simulink model "gm_comm8qamtxrxhdl"  (R2025b)
settings: Solver=FixedStepDiscrete  StartTime=0.0  StopTime=20000*qam_params.symbolPeriod  RelTol=1e-3
PreLoadFcn:
  | qam_params = comm8qamtxrxhdl_init;
InitFcn:
  | qam_params = comm8qamtxrxhdl_init;
libraries: simulink x16, hdlmdlgenlib x7, hdlsllib x7, commchan3 x1, commrflib2 x1, dspsigops x1, dsphdlsigops2 x1, dspmlti4 x1, commdigbbndam3 x1, commsequence2 x1
(part 3 of 3)

== system gm_comm8qamtxrxhdl/QAM Rx HDL/Coarse Frequency Offset Correction/Frequency Offset Estimation/Iteration ==
  xin : Inport  OutDataTypeStr=fixdt(1, 17, 13)  SampleTime=5e-07
  yin : Inport  Port=2  OutDataTypeStr=fixdt(1, 17, 13)  SampleTime=5e-07
  zin : Inport  Port=3  OutDataTypeStr=fixdt(1, 19, 18)  SampleTime=5e-07
  lut_value : Inport  Port=4  OutDataTypeStr=fixdt(0, 16, 18)  SampleTime=5e-07
  idx : Inport  Port=5  OutDataTypeStr=fixdt(0, 4, 0)  SampleTime=5e-07
  MuxX : Switch  Criteria=u2 ~= 0  Threshold="fi(0,0,1,0,\"hex\",\"0\")"  OutDataTypeStr=fixdt(1, 17, 13)  SampleTime=5e-07  SaturateOnIntegerOverflow=off  InputSameDT=off
  MuxY : Switch  Criteria=u2 ~= 0  Threshold="fi(0,0,1,0,\"hex\",\"0\")"  OutDataTypeStr=fixdt(1, 17, 13)  SampleTime=5e-07  SaturateOnIntegerOverflow=off  InputSameDT=off
  MuxZ : Switch  Criteria=u2 ~= 0  Threshold="fi(0,0,1,0,\"hex\",\"0\")"  OutDataTypeStr=fixdt(1, 19, 18)  SampleTime=5e-07  SaturateOnIntegerOverflow=off  InputSameDT=off
  XAdder : Sum  OutDataTypeStr=fixdt(1, 17, 13)  SampleTime=5e-07
  XSubtractor : Sum  Inputs=+-  OutDataTypeStr=fixdt(1, 17, 13)  AccumDataTypeStr=fixdt(1, 17, 13)  SampleTime=5e-07
  YAdder : Sum  OutDataTypeStr=fixdt(1, 17, 13)  SampleTime=5e-07
  YSub : Sum  Inputs=+-  OutDataTypeStr=fixdt(1, 17, 13)  AccumDataTypeStr=fixdt(1, 17, 13)  SampleTime=5e-07
  ZAdder : Sum  OutDataTypeStr=fixdt(1, 19, 18)  SampleTime=5e-07
  ZSub : Sum  Inputs=+-  OutDataTypeStr=fixdt(1, 19, 18)  AccumDataTypeStr=fixdt(1, 19, 18)  SampleTime=5e-07
  compare : simulink/Logic and Bit Operations/Compare To Constant  relop=<  const=double(0)  OutDataTypeStr=boolean
  dynamic_shift : ArithShift  BitShiftNumberSource=Input port  BitShiftDirection=Right
      settings: InputPortMap=u0,p1
  dynamic_shift1 : ArithShift  BitShiftNumberSource=Input port  BitShiftDirection=Right
      settings: InputPortMap=u0,p1
  xout : Outport  OutDataTypeStr=fixdt(1, 17, 13)  SampleTime=5e-07
  yout : Outport  Port=2  OutDataTypeStr=fixdt(1, 17, 13)  SampleTime=5e-07
  zout : Outport  Port=3  OutDataTypeStr=fixdt(1, 19, 18)  SampleTime=5e-07
  wires:
  yin/1 -> YSub/1, YAdder/1, dynamic_shift1/1, compare/1
  xin/1 -> XAdder/1, XSubtractor/1, dynamic_shift/1
  dynamic_shift1/1 -> XAdder/2, XSubtractor/2
  idx/1 -> dynamic_shift1/2, dynamic_shift/2
  lut_value/1 -> ZAdder/2, ZSub/2
  dynamic_shift/1 -> YSub/2, YAdder/2
  YAdder/1 -> MuxY/1
  zin/1 -> ZAdder/1, ZSub/1
  YSub/1 -> MuxY/3
  XSubtractor/1 -> MuxX/1
  compare/1 -> MuxZ/2, MuxY/2, MuxX/2
  XAdder/1 -> MuxX/3
  ZSub/1 -> MuxZ/1
  ZAdder/1 -> MuxZ/3
  MuxY/1 -> yout/1
  MuxX/1 -> xout/1
  MuxZ/1 -> zout/1

== system gm_comm8qamtxrxhdl/QAM Rx HDL/Coarse Frequency Offset Correction/Frequency Offset Estimation/Iteration1 ==
  xin : Inport  OutDataTypeStr=fixdt(1, 17, 13)  SampleTime=5e-07
  yin : Inport  Port=2  OutDataTypeStr=fixdt(1, 17, 13)  SampleTime=5e-07
  zin : Inport  Port=3  OutDataTypeStr=fixdt(1, 19, 18)  SampleTime=5e-07
  lut_value : Inport  Port=4  OutDataTypeStr=fixdt(0, 16, 18)  SampleTime=5e-07
  idx : Inport  Port=5  OutDataTypeStr=fixdt(0, 4, 0)  SampleTime=5e-07
  MuxX : Switch  Criteria=u2 ~= 0  Threshold="fi(0,0,1,0,\"hex\",\"0\")"  OutDataTypeStr=fixdt(1, 17, 13)  SampleTime=5e-07  SaturateOnIntegerOverflow=off  InputSameDT=off
  MuxY : Switch  Criteria=u2 ~= 0  Threshold="fi(0,0,1,0,\"hex\",\"0\")"  OutDataTypeStr=fixdt(1, 17, 13)  SampleTime=5e-07  SaturateOnIntegerOverflow=off  InputSameDT=off
  MuxZ : Switch  Criteria=u2 ~= 0  Threshold="fi(0,0,1,0,\"hex\",\"0\")"  OutDataTypeStr=fixdt(1, 19, 18)  SampleTime=5e-07  SaturateOnIntegerOverflow=off  InputSameDT=off
  XAdder : Sum  OutDataTypeStr=fixdt(1, 17, 13)  SampleTime=5e-07
  XSubtractor : Sum  Inputs=+-  OutDataTypeStr=fixdt(1, 17, 13)  AccumDataTypeStr=fixdt(1, 17, 13)  SampleTime=5e-07
  YAdder : Sum  OutDataTypeStr=fixdt(1, 17, 13)  SampleTime=5e-07
  YSub : Sum  Inputs=+-  OutDataTypeStr=fixdt(1, 17, 13)  AccumDataTypeStr=fixdt(1, 17, 13)  SampleTime=5e-07
  ZAdder : Sum  OutDataTypeStr=fixdt(1, 19, 18)  SampleTime=5e-07
  ZSub : Sum  Inputs=+-  OutDataTypeStr=fixdt(1, 19, 18)  AccumDataTypeStr=fixdt(1, 19, 18)  SampleTime=5e-07
  compare : simulink/Logic and Bit Operations/Compare To Constant  relop=<  const=double(0)  OutDataTypeStr=boolean
  dynamic_shift : ArithShift  BitShiftNumberSource=Input port  BitShiftDirection=Right
      settings: InputPortMap=u0,p1
  dynamic_shift1 : ArithShift  BitShiftNumberSource=Input port  BitShiftDirection=Right
      settings: InputPortMap=u0,p1
  xout : Outport  OutDataTypeStr=fixdt(1, 17, 13)  SampleTime=5e-07
  yout : Outport  Port=2  OutDataTypeStr=fixdt(1, 17, 13)  SampleTime=5e-07
  zout : Outport  Port=3  OutDataTypeStr=fixdt(1, 19, 18)  SampleTime=5e-07
  wires:
  yin/1 -> YAdder/1, YSub/1, dynamic_shift1/1, compare/1
  xin/1 -> XSubtractor/1, XAdder/1, dynamic_shift/1
  idx/1 -> dynamic_shift/2, dynamic_shift1/2
  zin/1 -> ZSub/1, ZAdder/1
  dynamic_shift/1 -> YSub/2, YAdder/2
  ZSub/1 -> MuxZ/1
  dynamic_shift1/1 -> XSubtractor/2, XAdder/2
  lut_value/1 -> ZSub/2, ZAdder/2
  ZAdder/1 -> MuxZ/3
  YAdder/1 -> MuxY/1
  compare/1 -> MuxX/2, MuxY/2, MuxZ/2
  YSub/1 -> MuxY/3
  XSubtractor/1 -> MuxX/1
  XAdder/1 -> MuxX/3
  MuxZ/1 -> zout/1
  MuxY/1 -> yout/1
  MuxX/1 -> xout/1

== system gm_comm8qamtxrxhdl/QAM Rx HDL/Coarse Frequency Offset Correction/Frequency Offset Estimation/Iteration2 ==
  xin : Inport  OutDataTypeStr=fixdt(1, 17, 13)  SampleTime=5e-07
  yin : Inport  Port=2  OutDataTypeStr=fixdt(1, 17, 13)  SampleTime=5e-07
  zin : Inport  Port=3  OutDataTypeStr=fixdt(1, 19, 18)  SampleTime=5e-07
  lut_value : Inport  Port=4  OutDataTypeStr=fixdt(0, 16, 18)  SampleTime=5e-07
  idx : Inport  Port=5  OutDataTypeStr=fixdt(0, 4, 0)  SampleTime=5e-07
  MuxX : Switch  Criteria=u2 ~= 0  Threshold="fi(0,0,1,0,\"hex\",\"0\")"  OutDataTypeStr=fixdt(1, 17, 13)  SampleTime=5e-07  SaturateOnIntegerOverflow=off  InputSameDT=off
  MuxY : Switch  Criteria=u2 ~= 0  Threshold="fi(0,0,1,0,\"hex\",\"0\")"  OutDataTypeStr=fixdt(1, 17, 13)  SampleTime=5e-07  SaturateOnIntegerOverflow=off  InputSameDT=off
  MuxZ : Switch  Criteria=u2 ~= 0  Threshold="fi(0,0,1,0,\"hex\",\"0\")"  OutDataTypeStr=fixdt(1, 19, 18)  SampleTime=5e-07  SaturateOnIntegerOverflow=off  InputSameDT=off
  XAdder : Sum  OutDataTypeStr=fixdt(1, 17, 13)  SampleTime=5e-07
  XSubtractor : Sum  Inputs=+-  OutDataTypeStr=fixdt(1, 17, 13)  AccumDataTypeStr=fixdt(1, 17, 13)  SampleTime=5e-07
  YAdder : Sum  OutDataTypeStr=fixdt(1, 17, 13)  SampleTime=5e-07
  YSub : Sum  Inputs=+-  OutDataTypeStr=fixdt(1, 17, 13)  AccumDataTypeStr=fixdt(1, 17, 13)  SampleTime=5e-07
  ZAdder : Sum  OutDataTypeStr=fixdt(1, 19, 18)  SampleTime=5e-07
  ZSub : Sum  Inputs=+-  OutDataTypeStr=fixdt(1, 19, 18)  AccumDataTypeStr=fixdt(1, 19, 18)  SampleTime=5e-07
  compare : simulink/Logic and Bit Operations/Compare To Constant  relop=<  const=double(0)  OutDataTypeStr=boolean
  dynamic_shift : ArithShift  BitShiftNumberSource=Input port  BitShiftDirection=Right
      settings: InputPortMap=u0,p1
  dynamic_shift1 : ArithShift  BitShiftNumberSource=Input port  BitShiftDirection=Right
      settings: InputPortMap=u0,p1
  xout : Outport  OutDataTypeStr=fixdt(1, 17, 13)  SampleTime=5e-07
  yout : Outport  Port=2  OutDataTypeStr=fixdt(1, 17, 13)  SampleTime=5e-07
  zout : Outport  Port=3  OutDataTypeStr=fixdt(1, 19, 18)  SampleTime=5e-07
  wires:
  dynamic_shift/1 -> YSub/2, YAdder/2
  yin/1 -> YSub/1, compare/1, YAdder/1, dynamic_shift1/1
  xin/1 -> XAdder/1, dynamic_shift/1, XSubtractor/1
  YAdder/1 -> MuxY/1
  idx/1 -> dynamic_shift1/2, dynamic_shift/2
  dynamic_shift1/1 -> XAdder/2, XSubtractor/2
  zin/1 -> ZAdder/1, ZSub/1
  lut_value/1 -> ZAdder/2, ZSub/2
  YSub/1 -> MuxY/3
  XSubtractor/1 -> MuxX/1
  compare/1 -> MuxZ/2, MuxY/2, MuxX/2
  XAdder/1 -> MuxX/3
  ZSub/1 -> MuxZ/1
  ZAdder/1 -> MuxZ/3
  MuxY/1 -> yout/1
  MuxX/1 -> xout/1
  MuxZ/1 -> zout/1

== system gm_comm8qamtxrxhdl/QAM Rx HDL/Coarse Frequency Offset Correction/Frequency Offset Estimation/Iteration3 ==
  xin : Inport  OutDataTypeStr=fixdt(1, 17, 13)  SampleTime=5e-07
  yin : Inport  Port=2  OutDataTypeStr=fixdt(1, 17, 13)  SampleTime=5e-07
  zin : Inport  Port=3  OutDataTypeStr=fixdt(1, 19, 18)  SampleTime=5e-07
  lut_value : Inport  Port=4  OutDataTypeStr=fixdt(0, 16, 18)  SampleTime=5e-07
  idx : Inport  Port=5  OutDataTypeStr=fixdt(0, 4, 0)  SampleTime=5e-07
  MuxX : Switch  Criteria=u2 ~= 0  Threshold="fi(0,0,1,0,\"hex\",\"0\")"  OutDataTypeStr=fixdt(1, 17, 13)  SampleTime=5e-07  SaturateOnIntegerOverflow=off  InputSameDT=off
  MuxY : Switch  Criteria=u2 ~= 0  Threshold="fi(0,0,1,0,\"hex\",\"0\")"  OutDataTypeStr=fixdt(1, 17, 13)  SampleTime=5e-07  SaturateOnIntegerOverflow=off  InputSameDT=off
  MuxZ : Switch  Criteria=u2 ~= 0  Threshold="fi(0,0,1,0,\"hex\",\"0\")"  OutDataTypeStr=fixdt(1, 19, 18)  SampleTime=5e-07  SaturateOnIntegerOverflow=off  InputSameDT=off
  XAdder : Sum  OutDataTypeStr=fixdt(1, 17, 13)  SampleTime=5e-07
  XSubtractor : Sum  Inputs=+-  OutDataTypeStr=fixdt(1, 17, 13)  AccumDataTypeStr=fixdt(1, 17, 13)  SampleTime=5e-07
  YAdder : Sum  OutDataTypeStr=fixdt(1, 17, 13)  SampleTime=5e-07
  YSub : Sum  Inputs=+-  OutDataTypeStr=fixdt(1, 17, 13)  AccumDataTypeStr=fixdt(1, 17, 13)  SampleTime=5e-07
  ZAdder : Sum  OutDataTypeStr=fixdt(1, 19, 18)  SampleTime=5e-07
  ZSub : Sum  Inputs=+-  OutDataTypeStr=fixdt(1, 19, 18)  AccumDataTypeStr=fixdt(1, 19, 18)  SampleTime=5e-07
  compare : simulink/Logic and Bit Operations/Compare To Constant  relop=<  const=double(0)  OutDataTypeStr=boolean
  dynamic_shift : ArithShift  BitShiftNumberSource=Input port  BitShiftDirection=Right
      settings: InputPortMap=u0,p1
  dynamic_shift1 : ArithShift  BitShiftNumberSource=Input port  BitShiftDirection=Right
      settings: InputPortMap=u0,p1
  xout : Outport  OutDataTypeStr=fixdt(1, 17, 13)  SampleTime=5e-07
  yout : Outport  Port=2  OutDataTypeStr=fixdt(1, 17, 13)  SampleTime=5e-07
  zout : Outport  Port=3  OutDataTypeStr=fixdt(1, 19, 18)  SampleTime=5e-07
  wires:
  lut_value/1 -> ZSub/2, ZAdder/2
  yin/1 -> compare/1, YAdder/1, YSub/1, dynamic_shift1/1
  xin/1 -> XSubtractor/1, dynamic_shift/1, XAdder/1
  idx/1 -> dynamic_shift/2, dynamic_shift1/2
  zin/1 -> ZAdder/1, ZSub/1
  dynamic_shift/1 -> YAdder/2, YSub/2
  ZSub/1 -> MuxZ/1
  dynamic_shift1/1 -> XSubtractor/2, XAdder/2
  ZAdder/1 -> MuxZ/3
  YAdder/1 -> MuxY/1
  compare/1 -> MuxY/2, MuxX/2, MuxZ/2
  YSub/1 -> MuxY/3
  XSubtractor/1 -> MuxX/1
  XAdder/1 -> MuxX/3
  MuxZ/1 -> zout/1
  MuxY/1 -> yout/1
  MuxX/1 -> xout/1

== system gm_comm8qamtxrxhdl/QAM Rx HDL/Coarse Frequency Offset Correction/Frequency Offset Estimation/Iteration4 ==
  xin : Inport  OutDataTypeStr=fixdt(1, 17, 13)  SampleTime=5e-07
  yin : Inport  Port=2  OutDataTypeStr=fixdt(1, 17, 13)  SampleTime=5e-07
  zin : Inport  Port=3  OutDataTypeStr=fixdt(1, 19, 18)  SampleTime=5e-07
  lut_value : Inport  Port=4  OutDataTypeStr=fixdt(0, 16, 18)  SampleTime=5e-07
  idx : Inport  Port=5  OutDataTypeStr=fixdt(0, 4, 0)  SampleTime=5e-07
  MuxX : Switch  Criteria=u2 ~= 0  Threshold="fi(0,0,1,0,\"hex\",\"0\")"  OutDataTypeStr=fixdt(1, 17, 13)  SampleTime=5e-07  SaturateOnIntegerOverflow=off  InputSameDT=off
  MuxY : Switch  Criteria=u2 ~= 0  Threshold="fi(0,0,1,0,\"hex\",\"0\")"  OutDataTypeStr=fixdt(1, 17, 13)  SampleTime=5e-07  SaturateOnIntegerOverflow=off  InputSameDT=off
  MuxZ : Switch  Criteria=u2 ~= 0  Threshold="fi(0,0,1,0,\"hex\",\"0\")"  OutDataTypeStr=fixdt(1, 19, 18)  SampleTime=5e-07  SaturateOnIntegerOverflow=off  InputSameDT=off
  XAdder : Sum  OutDataTypeStr=fixdt(1, 17, 13)  SampleTime=5e-07
  XSubtractor : Sum  Inputs=+-  OutDataTypeStr=fixdt(1, 17, 13)  AccumDataTypeStr=fixdt(1, 17, 13)  SampleTime=5e-07
  YAdder : Sum  OutDataTypeStr=fixdt(1, 17, 13)  SampleTime=5e-07
  YSub : Sum  Inputs=+-  OutDataTypeStr=fixdt(1, 17, 13)  AccumDataTypeStr=fixdt(1, 17, 13)  SampleTime=5e-07
  ZAdder : Sum  OutDataTypeStr=fixdt(1, 19, 18)  SampleTime=5e-07
  ZSub : Sum  Inputs=+-  OutDataTypeStr=fixdt(1, 19, 18)  AccumDataTypeStr=fixdt(1, 19, 18)  SampleTime=5e-07
  compare : simulink/Logic and Bit Operations/Compare To Constant  relop=<  const=double(0)  OutDataTypeStr=boolean
  dynamic_shift : ArithShift  BitShiftNumberSource=Input port  BitShiftDirection=Right
      settings: InputPortMap=u0,p1
  dynamic_shift1 : ArithShift  BitShiftNumberSource=Input port  BitShiftDirection=Right
      settings: InputPortMap=u0,p1
  xout : Outport  OutDataTypeStr=fixdt(1, 17, 13)  SampleTime=5e-07
  yout : Outport  Port=2  OutDataTypeStr=fixdt(1, 17, 13)  SampleTime=5e-07
  zout : Outport  Port=3  OutDataTypeStr=fixdt(1, 19, 18)  SampleTime=5e-07
  wires:
  yin/1 -> YSub/1, YAdder/1, compare/1, dynamic_shift1/1
  xin/1 -> XAdder/1, XSubtractor/1, dynamic_shift/1
  dynamic_shift1/1 -> XAdder/2, XSubtractor/2
  idx/1 -> dynamic_shift1/2, dynamic_shift/2
  zin/1 -> ZAdder/1, ZSub/1
  lut_value/1 -> ZAdder/2, ZSub/2
  dynamic_shift/1 -> YSub/2, YAdder/2
  YAdder/1 -> MuxY/1
  YSub/1 -> MuxY/3
  XSubtractor/1 -> MuxX/1
  compare/1 -> MuxY/2, MuxX/2, MuxZ/2
  XAdder/1 -> MuxX/3
  ZSub/1 -> MuxZ/1
  ZAdder/1 -> MuxZ/3
  MuxY/1 -> yout/1
  MuxX/1 -> xout/1
  MuxZ/1 -> zout/1

== system gm_comm8qamtxrxhdl/QAM Rx HDL/Coarse Frequency Offset Correction/Frequency Offset Estimation/QuadrantCorrection ==
  zin : Inport  OutDataTypeStr=fixdt(1, 19, 18)  SampleTime=5e-07
  QA_Control : Inport  Port=2  OutDataTypeStr=fixdt(0, 5, 0)  SampleTime=5e-07
  Negation : Gain  Gain="fi(0,1,2,0,\"hex\",\"3\")"  ParamDataTypeStr=fixdt(1, 2, 0)  OutDataTypeStr=fixdt(1, 19, 18)  SampleTime=5e-07
  adder : Sum  OutDataTypeStr=fixdt(1, 19, 18)  SampleTime=5e-07
  dtc : hdlmdlgenlib/Buffer
  extract : simulink/Logic and Bit Operations/Extract Bits  bitsToExtract=Range of bits  numBits=8  bitIdxRange=[2 2]  outScalingMode=Treat bit field as an integer
  extract1 : simulink/Logic and Bit Operations/Extract Bits  bitsToExtract=Range of bits  numBits=8  bitIdxRange=[0 1]  outScalingMode=Treat bit field as an integer
  mux : MultiPortSwitch  DataPortOrder=Zero-based contiguous  Inputs=2  DiagnosticForDefault=None  zeroidx=on  OutDataTypeStr=fixdt(1, 19, 18)  SampleTime=5e-07  SaturateOnIntegerOverflow=off  InputSameDT=off
  mux1 : MultiPortSwitch  DataPortOrder=Zero-based contiguous  Inputs=4  DiagnosticForDefault=None  zeroidx=on  OutDataTypeStr=fixdt(1, 19, 18)  SampleTime=5e-07  SaturateOnIntegerOverflow=off  InputSameDT=off
  mux2 : MultiPortSwitch  DataPortOrder=Zero-based contiguous  Inputs=2  DiagnosticForDefault=None  zeroidx=on  OutDataTypeStr=fixdt(1, 19, 18)  SampleTime=5e-07  SaturateOnIntegerOverflow=off  InputSameDT=off
  mux3 : MultiPortSwitch  DataPortOrder=Zero-based contiguous  Inputs=2  DiagnosticForDefault=None  zeroidx=on  OutDataTypeStr=fixdt(1, 19, 18)  SampleTime=5e-07  SaturateOnIntegerOverflow=off  InputSameDT=off
  mux6out_wire : hdlmdlgenlib/Buffer
  pidivtwoconstant : Constant  Value=0.5  OutDataTypeStr=fixdt(1, 19, 18)  SampleTime=5e-07
  pidivtwoconstant1 : Constant  Value=0.999996185302734375  OutDataTypeStr=fixdt(1, 19, 18)  SampleTime=5e-07
  pidivtwoconstant2 : Constant  Value=-1  OutDataTypeStr=fixdt(1, 19, 18)  SampleTime=5e-07
  pidivtwoconstant3 : Constant  Value=0  OutDataTypeStr=fixdt(1, 19, 18)  SampleTime=5e-07
  pidivtwosub : Sum  Inputs=+-  OutDataTypeStr=fixdt(1, 19, 18)  AccumDataTypeStr=fixdt(1, 19, 18)  SampleTime=5e-07
  slice : hdlsllib/Logic and Bit Operations/Bit Slice  lidx=double(3)  ridx=double(3)
  slice1 : hdlsllib/Logic and Bit Operations/Bit Slice  lidx=double(4)  ridx=double(4)
  subfmux : Sum  Inputs=+-  OutDataTypeStr=fixdt(1, 19, 18)  AccumDataTypeStr=fixdt(1, 19, 18)  SampleTime=5e-07
  zout : Outport  OutDataTypeStr=fixdt(1, 19, 18)  SampleTime=5e-07
  wires:
  mux3/1 -> mux6out_wire/1
  zin/1 -> dtc/1
  QA_Control/1 -> slice1/1, slice/1, extract1/1, extract/1
  pidivtwoconstant/1 -> pidivtwosub/1
  dtc/1 -> pidivtwosub/2, mux/3
  extract/1 -> mux/1
  extract1/1 -> mux1/1
  pidivtwosub/1 -> mux/2
  Negation/1 -> mux1/3
  mux/1 -> mux1/2, adder/2, subfmux/2, Negation/1
  pidivtwoconstant1/1 -> mux2/3, subfmux/1
  slice/1 -> mux2/1
  pidivtwoconstant2/1 -> adder/1
  subfmux/1 -> mux1/4
  adder/1 -> mux1/5
  slice1/1 -> mux3/1
  mux1/1 -> mux2/2
  mux2/1 -> mux3/2
  mux6out_wire/1 -> zout/1
  pidivtwoconstant3/1 -> mux3/3

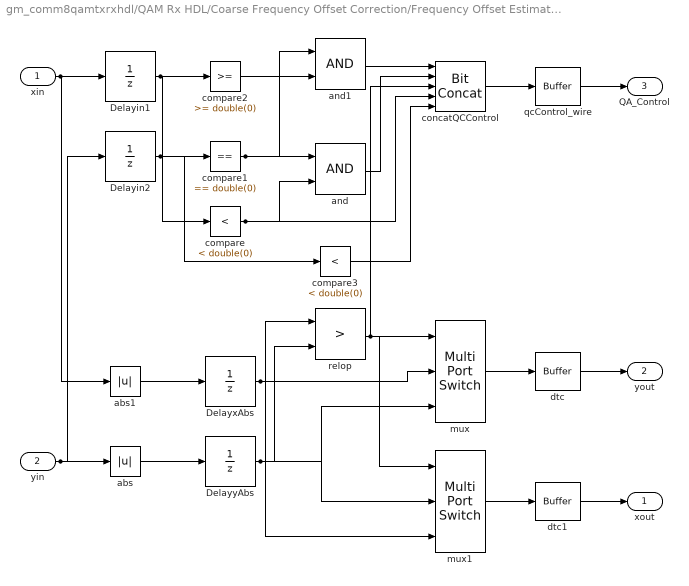
== system gm_comm8qamtxrxhdl/QAM Rx HDL/Coarse Frequency Offset Correction/Frequency Offset Estimation/QuadrantMapper ==
  xin : Inport  OutDataTypeStr=fixdt(1, 17, 13)  SampleTime=5e-07
  yin : Inport  Port=2  OutDataTypeStr=fixdt(1, 17, 13)  SampleTime=5e-07
  Delayin1 : UnitDelay  InitialCondition=double(0)  SampleTime=5e-07
  Delayin2 : UnitDelay  InitialCondition=double(0)  SampleTime=5e-07
  DelayxAbs : UnitDelay  InitialCondition=double(0)  SampleTime=5e-07
  DelayyAbs : UnitDelay  InitialCondition=double(0)  SampleTime=5e-07
  abs : Abs  SampleTime=5e-07  OutDataTypeStr=fixdt(1, 17, 13)  SaturateOnIntegerOverflow=off
  abs1 : Abs  SampleTime=5e-07  OutDataTypeStr=fixdt(1, 17, 13)  SaturateOnIntegerOverflow=off
  and : Logic  AllPortsSameDT=off  OutDataTypeStr=fixdt(0, 1, 0)  SampleTime=5e-07
  and1 : Logic  AllPortsSameDT=off  OutDataTypeStr=fixdt(0, 1, 0)  SampleTime=5e-07
  compare : simulink/Logic and Bit Operations/Compare To Constant  relop=<  const=double(0)  OutDataTypeStr=boolean
  compare1 : simulink/Logic and Bit Operations/Compare To Constant  relop===  const=double(0)  OutDataTypeStr=boolean
  compare2 : simulink/Logic and Bit Operations/Compare To Constant  relop=>=  const=double(0)  OutDataTypeStr=boolean
  compare3 : simulink/Logic and Bit Operations/Compare To Constant  relop=<  const=double(0)  OutDataTypeStr=boolean
  concatQCControl : hdlsllib/Logic and Bit Operations/Bit Concat  numInputs=5
  dtc : hdlmdlgenlib/Buffer
  dtc1 : hdlmdlgenlib/Buffer
  mux : MultiPortSwitch  DataPortOrder=Zero-based contiguous  Inputs=2  DiagnosticForDefault=None  zeroidx=on  OutDataTypeStr=fixdt(1, 17, 13)  SampleTime=5e-07  SaturateOnIntegerOverflow=off  InputSameDT=off
  mux1 : MultiPortSwitch  DataPortOrder=Zero-based contiguous  Inputs=2  DiagnosticForDefault=None  zeroidx=on  OutDataTypeStr=fixdt(1, 17, 13)  SampleTime=5e-07  SaturateOnIntegerOverflow=off  InputSameDT=off
  qcControl_wire : hdlmdlgenlib/Buffer
  relop : RelationalOperator  Operator=>  OutDataTypeStr=fixdt(0, 1, 0)  SampleTime=5e-07
  xout : Outport  OutDataTypeStr=fixdt(1, 17, 13)  SampleTime=5e-07
  yout : Outport  Port=2  OutDataTypeStr=fixdt(1, 17, 13)  SampleTime=5e-07
  QA_Control : Outport  Port=3  OutDataTypeStr=fixdt(0, 5, 0)  SampleTime=5e-07
  wires:
  Delayin2/1 -> compare3/1, compare1/1
  xin/1 -> abs1/1, Delayin1/1
  and/1 -> concatQCControl/2
  abs/1 -> DelayyAbs/1
  yin/1 -> Delayin2/1, abs/1
  Delayin1/1 -> compare/1, compare2/1
  compare1/1 -> and1/1, and/1
  and1/1 -> concatQCControl/1
  compare2/1 -> and1/2
  abs1/1 -> DelayxAbs/1
  compare/1 -> concatQCControl/4, and/2
  DelayxAbs/1 -> mux1/3, mux/2, relop/1
  DelayyAbs/1 -> mux1/2, relop/2, mux/3
  compare3/1 -> concatQCControl/5
  relop/1 -> concatQCControl/3, mux/1, mux1/1
  concatQCControl/1 -> qcControl_wire/1
  mux/1 -> dtc/1
  mux1/1 -> dtc1/1
  qcControl_wire/1 -> QA_Control/1
  dtc/1 -> yout/1
  dtc1/1 -> xout/1

== system gm_comm8qamtxrxhdl/QAM Rx HDL/Coarse Frequency Offset Correction/Frequency Offset Estimation/Raise to Power 4 ==
  In1 : Inport  OutDataTypeStr=fixdt(1, 16, 15)  PortDimensions=1  SampleTime=5e-07
      settings: SignalType=complex
  Delay1 : Delay  DelayLength=double(2)  InitialCondition=0  SampleTime=5e-07
  Delay4 : Delay  DelayLength=double(4)  InitialCondition=0  SampleTime=5e-07
  Delay5 : Delay  DelayLength=double(4)  InitialCondition=0  SampleTime=5e-07
  Product : Product  Inputs=**  OutDataTypeStr=fixdt(1, 16, 15)  SampleTime=5e-07
  Product1 : Product  Inputs=**  OutDataTypeStr=fixdt(1, 16, 15)  SampleTime=5e-07
  Out1 : Outport  SampleTime=5e-07  VectorParamsAs1DForOutWhenUnconnected=off
  wires:
  In1/1 -> Delay1/1
  Delay1/1 -> Product/1, Product/2
  Product/1 -> Delay4/1
  Delay4/1 -> Product1/1, Product1/2
  Product1/1 -> Delay5/1
  Delay5/1 -> Out1/1

== system gm_comm8qamtxrxhdl/QAM Rx HDL/Magnitude & Phase Recovery/MATLAB Function3/MATLAB Function3 ==
  enable : Inport  OutDataTypeStr=boolean  PortDimensions=1  SampleTime=5e-07
  MATLAB Function3 : MATLAB Function  TreatAsAtomicUnit=on
  dvalid : Outport  SampleTime=5e-07  VectorParamsAs1DForOutWhenUnconnected=off
  isPreamble : Outport  Port=2  SampleTime=5e-07  VectorParamsAs1DForOutWhenUnconnected=off
  wires:
  MATLAB Function3/2(isPreamble) -> isPreamble/1
  MATLAB Function3/1(dvalid) -> dvalid/1
  enable/1 -> MATLAB Function3/1(enable)

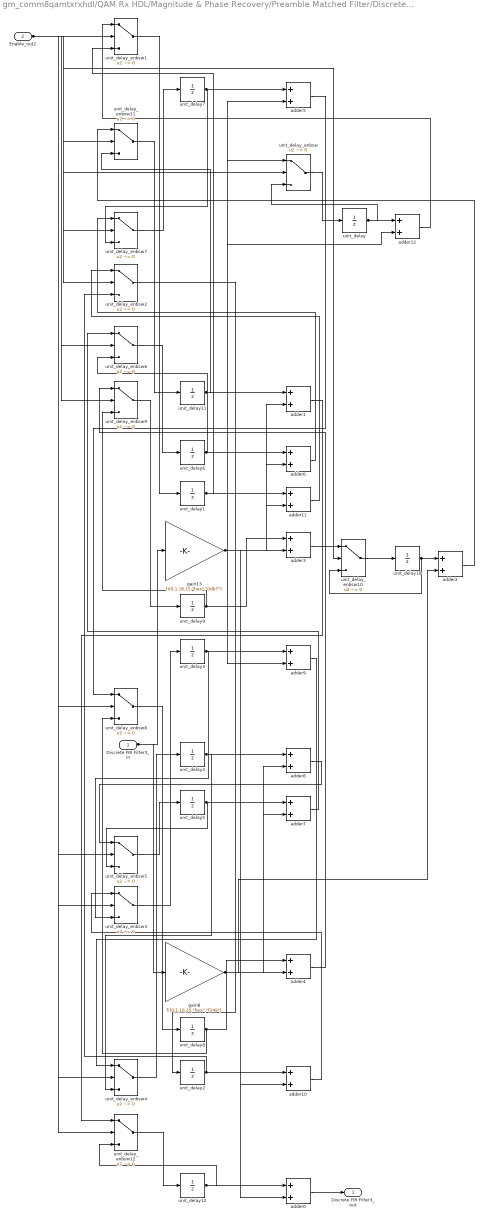
== system gm_comm8qamtxrxhdl/QAM Rx HDL/Magnitude & Phase Recovery/Preamble Matched Filter/Discrete FIR Filter3 ==
  Discrete FIR Filter3_in : Inport  OutDataTypeStr=fixdt(1, 17, 15)  SampleTime=5e-07
  Enable_out2 : Inport  Port=2  OutDataTypeStr=boolean  SampleTime=5e-07
  adder{0..12} (13 alike) : Sum  OutDataTypeStr=fixdt(1, 17, 15)  SampleTime=5e-07
  gain13 : Gain  Gain="fi(0,1,16,15,\"hex\",\"0db7\")"  ParamDataTypeStr=fixdt(1, 16, 15)  OutDataTypeStr=fixdt(1, 16, 15)  SampleTime=5e-07
  gain8 : Gain  Gain="fi(0,1,16,15,\"hex\",\"f249\")"  ParamDataTypeStr=fixdt(1, 16, 15)  OutDataTypeStr=fixdt(1, 16, 15)  SampleTime=5e-07
  unit_delay{,1..12} (13 alike) : UnitDelay  InitialCondition=double(0)  SampleTime=5e-07
  unit_delay_enbsw : Switch  Criteria=u2 ~= 0  Threshold=double(0)  OutDataTypeStr=fixdt(1, 16, 15)  SampleTime=5e-07  SaturateOnIntegerOverflow=off  InputSameDT=off
  unit_delay_enbsw{1..12} (12 alike) : Switch  Criteria=u2 ~= 0  Threshold=double(0)  OutDataTypeStr=fixdt(1, 17, 15)  SampleTime=5e-07  SaturateOnIntegerOverflow=off  InputSameDT=off
  Discrete FIR Filter3_out : Outport  OutDataTypeStr=fixdt(1, 17, 15)  SampleTime=5e-07
  wires:
  unit_delay_enbsw6/1 -> unit_delay6/1
  gain8/1 -> adder2/2, adder4/2, adder7/2, adder8/2
  unit_delay_enbsw2/1 -> unit_delay2/1
  Enable_out2/1 -> unit_delay_enbsw2/2, unit_delay_enbsw9/2, unit_delay_enbsw1/2, unit_delay_enbsw3/2, unit_delay_enbsw6/2, unit_delay_enbsw8/2, unit_delay_enbsw7/2, unit_delay_enbsw5/2, unit_delay_enbsw10/2, unit_delay_enbsw4/2, unit_delay_enbsw11/2, unit_delay_enbsw12/2, unit_delay_enbsw/2
  unit_delay_enbsw9/1 -> unit_delay9/1
  adder1/1 -> unit_delay_enbsw12/1
  unit_delay_enbsw1/1 -> unit_delay1/1
  unit_delay_enbsw7/1 -> unit_delay7/1
  unit_delay_enbsw11/1 -> unit_delay11/1
  unit_delay_enbsw8/1 -> unit_delay8/1
  unit_delay6/1 -> unit_delay_enbsw6/3, adder6/1
  Discrete FIR Filter3_in/1 -> gain13/1, gain8/1
  unit_delay_enbsw5/1 -> unit_delay5/1
  unit_delay_enbsw3/1 -> unit_delay3/1
  unit_delay_enbsw4/1 -> unit_delay4/1
  unit_delay_enbsw12/1 -> unit_delay12/1
  unit_delay7/1 -> adder5/1, unit_delay_enbsw7/3
  unit_delay11/1 -> unit_delay_enbsw11/3, adder1/1
  unit_delay1/1 -> unit_delay_enbsw1/3, adder11/1
  gain13/1 -> adder12/2, adder0/2, adder3/2, adder5/2, adder6/2, adder11/2, adder10/2, unit_delay_enbsw/1, adder9/2, adder1/2
  unit_delay9/1 -> unit_delay_enbsw9/3, adder3/1
  unit_delay3/1 -> unit_delay_enbsw3/3, adder9/1
  unit_delay4/1 -> unit_delay_enbsw4/3, adder8/1
  unit_delay5/1 -> unit_delay_enbsw5/3, adder7/1
  unit_delay8/1 -> unit_delay_enbsw8/3, adder4/1
  adder0/1 -> Discrete FIR Filter3_out/1
  unit_delay2/1 -> unit_delay_enbsw2/3, adder10/1
  unit_delay12/1 -> unit_delay_enbsw12/3, adder0/1
  adder5/1 -> unit_delay_enbsw8/1
  unit_delay_enbsw/1 -> unit_delay/1
  adder6/1 -> unit_delay_enbsw7/1
  adder11/1 -> unit_delay_enbsw2/1
  adder3/1 -> unit_delay_enbsw10/1
  adder4/1 -> unit_delay_enbsw9/1
  adder9/1 -> unit_delay_enbsw4/1
  adder8/1 -> unit_delay_enbsw5/1
  adder7/1 -> unit_delay_enbsw6/1
  adder10/1 -> unit_delay_enbsw3/1
  unit_delay/1 -> unit_delay_enbsw/3, adder12/1
  unit_delay_enbsw10/1 -> unit_delay10/1
  adder12/1 -> unit_delay_enbsw1/1
  unit_delay10/1 -> unit_delay_enbsw10/3, adder2/1
  adder2/1 -> unit_delay_enbsw11/1

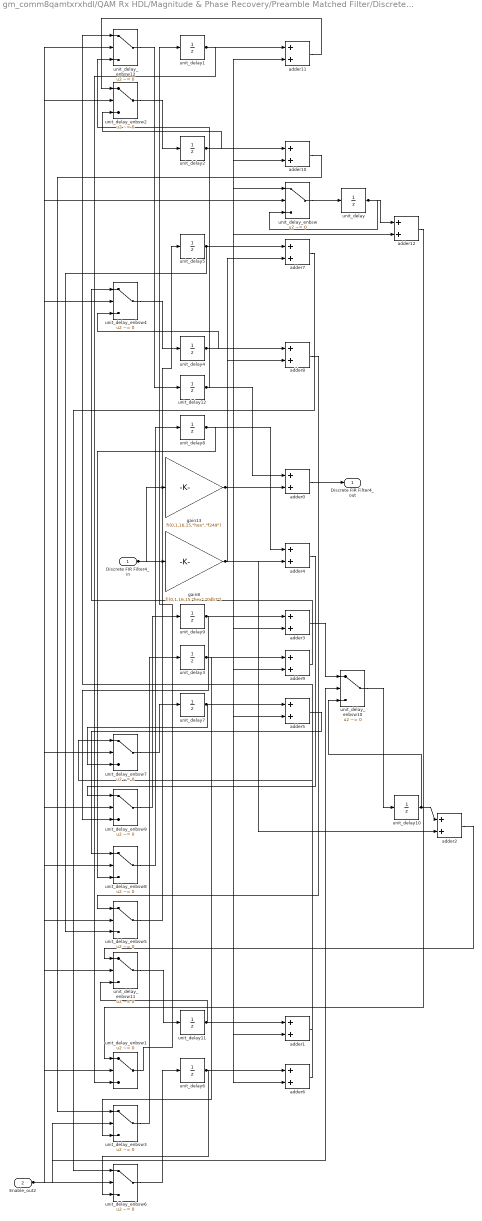
== system gm_comm8qamtxrxhdl/QAM Rx HDL/Magnitude & Phase Recovery/Preamble Matched Filter/Discrete FIR Filter4 ==
  Discrete FIR Filter4_in : Inport  OutDataTypeStr=fixdt(1, 17, 15)  SampleTime=5e-07
  Enable_out2 : Inport  Port=2  OutDataTypeStr=boolean  SampleTime=5e-07
  adder{0..12} (13 alike) : Sum  OutDataTypeStr=fixdt(1, 17, 15)  SampleTime=5e-07
  gain13 : Gain  Gain="fi(0,1,16,15,\"hex\",\"f249\")"  ParamDataTypeStr=fixdt(1, 16, 15)  OutDataTypeStr=fixdt(1, 16, 15)  SampleTime=5e-07
  gain8 : Gain  Gain="fi(0,1,16,15,\"hex\",\"0db7\")"  ParamDataTypeStr=fixdt(1, 16, 15)  OutDataTypeStr=fixdt(1, 16, 15)  SampleTime=5e-07
  unit_delay{,1..12} (13 alike) : UnitDelay  InitialCondition=double(0)  SampleTime=5e-07
  unit_delay_enbsw : Switch  Criteria=u2 ~= 0  Threshold=double(0)  OutDataTypeStr=fixdt(1, 16, 15)  SampleTime=5e-07  SaturateOnIntegerOverflow=off  InputSameDT=off
  unit_delay_enbsw{1..12} (12 alike) : Switch  Criteria=u2 ~= 0  Threshold=double(0)  OutDataTypeStr=fixdt(1, 17, 15)  SampleTime=5e-07  SaturateOnIntegerOverflow=off  InputSameDT=off
  Discrete FIR Filter4_out : Outport  OutDataTypeStr=fixdt(1, 17, 15)  SampleTime=5e-07
  wires:
  unit_delay_enbsw1/1 -> unit_delay1/1
  unit_delay_enbsw7/1 -> unit_delay7/1
  Enable_out2/1 -> unit_delay_enbsw1/2, unit_delay_enbsw3/2, unit_delay_enbsw4/2, unit_delay_enbsw6/2, unit_delay_enbsw7/2, unit_delay_enbsw9/2, unit_delay_enbsw5/2, unit_delay_enbsw8/2, unit_delay_enbsw11/2, unit_delay_enbsw2/2, unit_delay_enbsw10/2, unit_delay_enbsw12/2, unit_delay_enbsw/2
  unit_delay_enbsw8/1 -> unit_delay8/1
  unit_delay_enbsw4/1 -> unit_delay4/1
  unit_delay_enbsw2/1 -> unit_delay2/1
  adder0/1 -> Discrete FIR Filter4_out/1
  unit_delay_enbsw12/1 -> unit_delay12/1
  Discrete FIR Filter4_in/1 -> gain13/1, gain8/1
  unit_delay_enbsw3/1 -> unit_delay3/1
  unit_delay_enbsw9/1 -> unit_delay9/1
  unit_delay_enbsw5/1 -> unit_delay5/1
  unit_delay_enbsw11/1 -> unit_delay11/1
  unit_delay_enbsw6/1 -> unit_delay6/1
  unit_delay1/1 -> unit_delay_enbsw1/3, adder11/1
  unit_delay2/1 -> unit_delay_enbsw2/3, adder10/1
  adder9/1 -> unit_delay_enbsw4/1
  unit_delay5/1 -> unit_delay_enbsw5/3, adder7/1
  unit_delay4/1 -> unit_delay_enbsw4/3, adder8/1
  unit_delay12/1 -> unit_delay_enbsw12/3, adder0/1
  unit_delay8/1 -> unit_delay_enbsw8/3, adder4/1
  unit_delay6/1 -> unit_delay_enbsw6/3, adder6/1
  gain13/1 -> adder12/2, adder0/2, adder1/2, adder6/2, adder9/2, adder10/2, adder11/2, unit_delay_enbsw/1, adder3/2, adder5/2
  adder8/1 -> unit_delay_enbsw5/1
  gain8/1 -> adder7/2, adder4/2, adder8/2, adder2/2
  unit_delay9/1 -> unit_delay_enbsw9/3, adder3/1
  adder11/1 -> unit_delay_enbsw2/1
  unit_delay3/1 -> unit_delay_enbsw3/3, adder9/1
  unit_delay7/1 -> unit_delay_enbsw7/3, adder5/1
  unit_delay11/1 -> unit_delay_enbsw11/3, adder1/1
  adder10/1 -> unit_delay_enbsw3/1
  unit_delay_enbsw/1 -> unit_delay/1
  unit_delay_enbsw10/1 -> unit_delay10/1
  adder7/1 -> unit_delay_enbsw6/1
  adder4/1 -> unit_delay_enbsw9/1
  adder3/1 -> unit_delay_enbsw10/1
  adder5/1 -> unit_delay_enbsw8/1
  adder1/1 -> unit_delay_enbsw12/1
  adder6/1 -> unit_delay_enbsw7/1
  unit_delay/1 -> unit_delay_enbsw/3, adder12/1
  adder12/1 -> unit_delay_enbsw1/1
  unit_delay10/1 -> unit_delay_enbsw10/3, adder2/1
  adder2/1 -> unit_delay_enbsw11/1

== system gm_comm8qamtxrxhdl/QAM Tx HDL/Data Generation & Packetization/Data Source/HDL Data Scrambler ==
  note: HDL optimized scrambler, implementing the scrambler polynomial [1 1 1 0 1],
      |  with initial states [0 0 0 0]
  Data_In : Inport
  Enable : EnablePort
  BIT_XOR : Logic  Operator=XOR  IconShape=distinctive  AllPortsSameDT=off  OutDataTypeStr=boolean
  BIT_XOR1 : Logic  Operator=XOR  IconShape=distinctive  AllPortsSameDT=off  OutDataTypeStr=boolean
  BIT_XOR2 : Logic  Operator=XOR  IconShape=distinctive  AllPortsSameDT=off  OutDataTypeStr=boolean
  p{1..4} (4 alike) : Delay  DelayLength=1
  Scrambled_Out : Outport  InitialOutput=0  VectorParamsAs1DForOutWhenUnconnected=off
  wires:
  Data_In/1 -> BIT_XOR2/1
  BIT_XOR1/1 -> BIT_XOR2/2
  p2/1 -> p3/1, BIT_XOR/1
  p3/1 -> p4/1
  BIT_XOR/1 -> BIT_XOR1/2
  p1/1 -> BIT_XOR1/1, p2/1
  p4/1 -> BIT_XOR/2
  BIT_XOR2/1 -> p1/1, Scrambled_Out/1

== matlab function gm_comm8qamtxrxhdl/QAM Rx HDL/Timing Recovery/Interpolation Control/Interpolation Control ==
  data: Delta input; Underflow output; mu output
function [Underflow, mu] = Interpolation_ctrl(Delta)
% Implementation of modulo-1 counter for interpolation control listed in
% Figure 8.4.19 of "Digital Communications - A Discrete-Time Approach"
% by Michael Rice. See design details in Chapter 8.4.3 of the same book.
% 
% Input:
%   Delta - Loop filter output. If loop is in lock, delta would be small
% Output:
%   Underflow - Indicator of counter underflow. This is the strobe signal
%               for downstream processing
%   mu - Difference between actual sampling instant and the optimal instant,
%        between zero and one
%#codegen

% delay1 - Counter value delayed by 1 sample
% Regtemp - The estimated timing error normalized by half QPSK symbols

W = 16; % accumulator wordlength
F = 15; % accumulator fraction length

persistent delay1 Regtemp;  
if isempty(delay1)
    delay1  = fi(0,1,W,F);
    Regtemp = fi(0,1,W,F);
end

mask = fi(1-2^(-F),1,W,F);

counter = bitand(mask,delay1)-Delta-fi(0.5,1,W,F); % decrementing counter
% if delay1 is a nonnegative number,
% then mod(delay1,1) equals the fractional part of delay1

if counter < 0
    Underflow = true;
    Regtemp = bitshift(bitand(mask,delay1),1);     
else
    Underflow = false;
end

mu = Regtemp;

% Update delay buffer
% delay1 = counter;
if counter<0
    delay1 = fi(counter+1,1,W,F); %make sure delay1 is nonnegative
else
    delay1 = fi(counter,1,W,F);
end

== matlab function gm_comm8qamtxrxhdl/QAM Rx HDL/Timing Recovery/Timing Error Detector/Timing Error Detector ==
  data: In input; strobe input; e output
function e = TED(In, strobe)
% Zero-Crossing Timing Error Detector. See "Zero-Crossing Timing Error
% Detector" section in Chapter 8.4.1 of "Digital Communications - A
% Discrete-Time Approach" by Michael Rice. For bit stuffing/stripping
% details, see page 490-494 of the same book.
%
% Input: 
%   In - Input samples, interpolation result
%   strobe - Signal to enable timing error calculation
% Output:
%   e - Timing error
%#codegen

persistent delay1_R delay1_I delay2_R delay2_I delayStrobe; 
% Input delayed by one and 2 samples, and
% Enable signal delayed by one sample
if isempty(delay1_R)    
    delay1_R=fi(0,1,16,15);
    delay1_I=fi(0,1,16,15);
    delay2_R=fi(0,1,16,15);
    delay2_I=fi(0,1,16,15);    
    delayStrobe = false;
end

In_Real = real(In);
In_Imag = imag(In);

if strobe==true && delayStrobe~=strobe
    if ( bitget(delay2_R,16)==bitget(In_Real,16) )         
        OP1=fi(0,1,16,15);
    elseif bitget(delay2_R,16)==true         
        OP1=fi(-1*bitshift(delay1_R,1),1,16,15);
    else        
        OP1=fi(bitshift(delay1_R,1),1,16,15);
    end
    
    if ( bitget(delay2_I,16)==bitget(In_Imag,16) )        
        OP2=fi(0,1,16,15);
    elseif bitget(delay2_I,16)==true        
        OP2=fi(-1*bitshift(delay1_I,1),1,16,15);
    else        
        OP2=fi(bitshift(delay1_I,1),1,16,15);
    end
else
    OP1=fi(0,1,16,15);
    OP2=fi(0,1,16,15);
end

e = fi(OP1+OP2,1,16,15);


if delayStrobe~=strobe
    % Shift contents in delay register
    delay2_R = delay1_R;
    delay1_R = In_Real;
    delay2_I = delay1_I;
    delay1_I = In_Imag;
elseif strobe==true
    % Two consecutive high strobes
    delay2_R = fi(0,1,16,15); % Stuff missing sample
    delay1_R = In_Real; 
    delay2_I = fi(0,1,16,15); % Stuff missing sample
    delay1_I = In_Imag; 
end

% If both current and previous enable signals are 0, skip current sample
% and keep the delayed signals unchanged. (Bit stripping)
delayStrobe = strobe;

== matlab function gm_comm8qamtxrxhdl/QAM Rx HDL/Demodulate/Rectangular QAM Demodulator Baseband/Rectangular QAM Demodulator Baseband ==
  data: u input; y output
function y = Rect8QAMDemod(u)
%#codegen
% HDL-compatible Gray-coded 8-QAM Hard-Decision Demodulator (MinDist = 2)
% Constellation points: I in {-3, -1, +1, +3}, Q in {-1, +1}
I = real(u);
Q = imag(u);
b1 = (I >= 0);       % MSB: 0 for I < 0, 1 for I >= 0
b2 = (abs(I) <= 2);  % Mid: 0 for |I| > 2 (+-3), 1 for |I| <= 2 (+-1)
b3 = (Q < 0);        % LSB: 0 for Q >= 0 (+1), 1 for Q < 0 (-1)
y  = [b1; b2; b3];

== matlab function gm_comm8qamtxrxhdl/QAM Tx HDL/Data Generation & Packetization/Controller FSM ==
  data: reset_preamble output; load_preamble output; load_data output
function [reset_preamble,load_preamble, load_data] = ControllerFSM()
%#codegen

persistent packState;
persistent stateCounter;

sType = numerictype(0,1,0);
cType = numerictype(0,8,0);

if isempty(packState)
    packState = fi(0,'numerictype',sType);
    stateCounter  = fi(0,'numerictype',cType);
end

Pack_Preamble = fi(0,'numerictype',sType);
Append_Data   = fi(1,'numerictype',sType);

switch(packState)
    case Pack_Preamble  %% Pack_Preamble
        load_preamble  = true;
        reset_preamble = false;
        load_data      = false;
        
        if stateCounter == 41;  %% Pack_Preamble complete
            packState(:) = 1;                   %% move to Append_Data state
            stateCounter(:) = 0;                %% reset counter
        else
            packState(:) = 0;                   %% remain in Pack_Preamble state
            stateCounter(:) = stateCounter +1;  %% increment preamble count
        end
        
    case Append_Data    %% Append_Data
        load_preamble  = false;
        reset_preamble = true;
        load_data      = true;
        
        if stateCounter == 125  %% Append_Data complete
            packState(:) = 0;                   %% move to Pack_Preamble state
            stateCounter(:) = 0;                %% reset counter
        else
            packState(:) = 1;                   %% remain in Append_Data state
            stateCounter(:) = stateCounter +1;  %% increment data count
        end
        
    otherwise
        load_preamble  = false;
        reset_preamble = false;
        load_data      = false;
        stateCounter(:) = 0;
end

== matlab function gm_comm8qamtxrxhdl/Text Message Decoding/  ==
  data: newPacket input; dValid input; RxGo output; framed_data output; bit1 input; bit2 input; bit3 input
function [RxGo,framed_data] = dataframer(newPacket, dValid, bit1, bit2, bit3)
%#codegen

persistent gooddata_so_far frame_index

if isempty(gooddata_so_far)
    gooddata_so_far = false(168,1);
    frame_index = 1;
end

RxGo = false;
framed_data = false(168,1);

if dValid==true
    gooddata_so_far(frame_index:frame_index+2) = [bit1 bit2 bit3];
    frame_index = frame_index+3;
    if (frame_index==169) || (newPacket==true)
        RxGo = true;
        framed_data = gooddata_so_far;
        frame_index = 1;
    end
end

== matlab function gm_comm8qamtxrxhdl/QAM Rx HDL/Magnitude & Phase Recovery/MATLAB Function3/MATLAB Function3/MATLAB Function3 ==
  data: dvalid output; enable input; isPreamble output
function [dvalid,isPreamble] = fcn(enable)
%#codegen

persistent state;
persistent counter;


if isempty(state);
    state      = false;
    counter    = uint8(0);
end


if counter > 42
    isPreamble = true;
else
    isPreamble = false;
end


if state==false
    dvalid=false;
else %state==true
    dvalid=true;
    counter = counter-1;
end


% state transition
if state==false && enable==true
    state=true;
    counter=uint8(56);
elseif state==true && counter==0
    if enable==true % packages come back-to-back
        state      = true;
        counter    = uint8(56);
    else
        state = false;    
    end
end

== matlab function gm_comm8qamtxrxhdl/Text Message Decoding/Descramble and Print/BitsToDecimal1 ==
  data: u input
function BitsToASCII(u)
% Convert bits to ASCII message (8-QAM Option A: 18 chars = 126 bits).

persistent package_counter;
persistent error_counter;
if isempty(package_counter)
    package_counter = 0;
    error_counter   = 0;
end

coder.extrinsic('disp')
coder.extrinsic('num2str')

aa = de2bi(int8('Hello! ~8-QAM~ 0'),7,'left-msb');
bits_ref = double(reshape(aa.',1,[]));
bits_ref = bits_ref(:);

error_counter   = error_counter   + sum(abs(bits_ref - u(1:112)));
package_counter = package_counter + 1;

% Convert binary-valued column vector to 7-bit decimal values.
w = [64 32 16 8 4 2 1]; % binary digit weighting
Nbits = numel(u);
Ny = Nbits/7;
y = zeros(1,Ny);
for i = 0:Ny-1
    y(i+1) = w*u(7*i+(1:7));
end

% Display ASCII message to command window
if rem(package_counter,50)==0
    disp([char(y) '    ==>    BER = ' num2str(error_counter/50/7/16)]);
    error_counter = 0;
else
    disp(char(y));
end
